simulink model "Controller"  (R2026b)
settings: Solver=VariableStepAuto  StopTime=1200  MaxStep=0.1
values from neighbouring files (symbols this model uses):
  Hoffch = 0.5    [export_ref.m]    (also in init_params.m = 3; testseq.m)
  Honch = 0.5    [export_ref.m]    (also in init_params.m = 3; testseq.m)
  Kich = 6    [init_params.m]
  Kpch = 3000    [init_params.m]
  Ktch = 0.005    [init_params.m]
  Qmax = 24000    [init_params.m]
  Qmin = Qmax/turndown    (= 2400)    [init_params.m]
  Tsch = 0.1    [init_params.m]
undefined symbols (not defined in the file or in its folder): Kbch
libraries: slpidlib x1
settings Model: Creator=Ogun Serif  LastModifiedBy=Ogun Serif
settings DataIOCC: SaveOutput=off  SaveTime=off

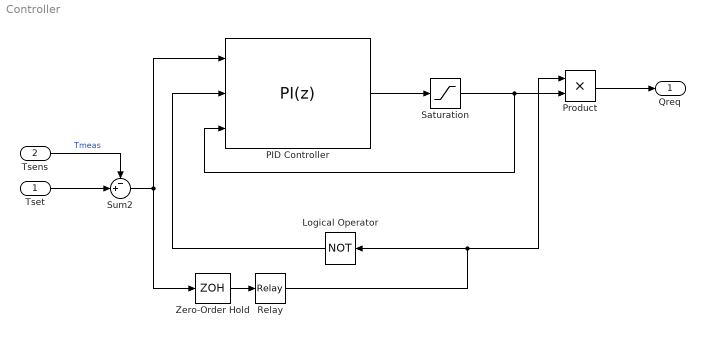
== system Controller ==
  Tset : Inport  OutDataTypeStr=double  PortDimensions=1
  Tsens : Inport  Port=2  OutDataTypeStr=double  PortDimensions=1  SampleTime=0
  Logical Operator : Logic  Operator=NOT  AllPortsSameDT=off  OutDataTypeStr=boolean
  PID Controller : slpidlib/PID Controller  Controller=PI  Form=Parallel  TimeDomain=Discrete-time  UseExternalTs=off  SampleTime=Tsch  IntegratorMethod=Forward Euler  FilterMethod=Forward Euler  ControllerParametersSource=internal  P=Kpch  I=Kich  UseKiTs=off  D=0  UseExternalDerivativeSource=off  N=100  UseFilter=on  TunerSelectOption=Transfer Function Based (PID Tuner App)  InitialConditionSource=internal  InitialConditionForIntegrator=0  InitialConditionForFilter=0  DifferentiatorICPrevScaledInput=0  ExternalReset=level  TrackingMode=on  Kt=Ktch  LimitOutput=off  SatLimitsSource=internal  UpperSaturationLimit=24000  LowerSaturationLimit=Qmin  LinearizeAsGain=on  AntiWindupMode=back-calculation  Kb=Kbch  LimitIntegrator=off  UpperIntegratorSaturationLimit=inf  LowerIntegratorSaturationLimit=-inf  POutMin=[]  POutMax=[]  IOutMin=[]  IOutMax=[]  DOutMin=[]  DOutMax=[]  NOutMin=[]  NOutMax=[]  SumOutMin=[]  SumOutMax=[]  SaturationOutMin=[]  SaturationOutMax=[]  PParamMin=[]  PParamMax=[]  IParamMin=[]  IParamMax=[]  DParamMin=[]  DParamMax=[]  NParamMin=[]  NParamMax=[]  KbParamMin=[]  KbParamMax=[]  KtParamMin=[]  KtParamMax=[]  KbOutMin=[]  KbOutMax=[]  KtOutMin=[]  KtOutMax=[]  IntegratorOutMin=[]  IntegratorOutMax=[]  FilterOutMin=[]  FilterOutMax=[]  SumI1OutMin=[]  SumI1OutMax=[]  SumI2OutMin=[]  SumI2OutMax=[]  SumI3OutMin=[]  SumI3OutMax=[]  SumI4OutMin=[]  SumI4OutMax=[]  SumDOutMin=[]  SumDOutMax=[]  DifferentiatorOutMin=[]  DifferentiatorOutMax=[]  FilterDiffOutCoefMin=[]  FilterDiffOutCoefMax=[]  ReciprocalOutMin=[]  ReciprocalOutMax=[]  SumDenOutMin=[]  SumDenOutMax=[]  SumNumOutMin=[]  SumNumOutMax=[]  DivideOutMin=[]  DivideOutMax=[]  UdiffTsProdOutMin=[]  UdiffTsProdOutMax=[]  NTsProdOutMin=[]  NTsProdOutMax=[]  UintegralTsProdOutMin=[]  UintegralTsProdOutMax=[]  UngainTsProdOutMin=[]  UngainTsProdOutMax=[]  ClampingZeroOutDataTypeStr=Inherit: Inherit via back propagation  ClampingZeroOutMin=[]  ClampingZeroOutMax=[]  FilterDenConstantOutDataTypeStr=Inherit: Inherit via back propagation  FilterDenConstantOutMin=[]  FilterDenConstantOutMax=[]  PCopyOutDataTypeStr=Inherit: Inherit via back propagation  PCopyOutMin=[]  PCopyOutMax=[]  NCopyOutDataTypeStr=Inherit: Inherit via back propagation  NCopyOutMin=[]  NCopyOutMax=[]  IntegratorContinuousStateAttributes=''  IntegratorStateMustResolveToSignalObject=off  IntegratorRTWStateStorageClass=Auto  FilterContinuousStateAttributes=''  FilterStateMustResolveToSignalObject=off  FilterRTWStateStorageClass=Auto  ParallelPVariant=InternalParameters  IdealPVariant=Disabled  IVariant=InternalParameters  DVariant=Disabled  IntegratorVariant=Discrete  SatVariant=Disabled  AWVariant=Passthrough  PCopyVariant=Disabled  TRVariant=Enabled  FdbkBlocksVariant=Forward  IdealPFdbkVariant=Disabled  SatFdbkVariant=Disabled  DerivativeFilterVariant=Disabled  NVariant=Disabled  NCopyVariant=Disabled_SignalSpec  FilterICVariant=Disabled  IntegratorICVariant=InternalICs  ExternalResetVariant=ExternalReset  TRSumVariant=TrackingMode  SumFdbkVariant=Disabled  SumVariant=Sum_PI  TsampFilterVariant=InternalTs  TsampNgainVariant=Passthrough  TsampIntegralVariant=Disabled_SignalSpec  ExternalSaturationOutDataTypeStr=Inherit: Same as second input  DerivativeSourceVariant=Disabled  PreIntVariant=InternalPreInt
  Product : Product
  Relay : Relay  OnSwitchValue=Honch  OffSwitchValue=-Hoffch
  Saturation : Saturate  UpperLimit=Qmax  LowerLimit=Qmin
  Sum2 : Sum  Inputs=-+|
  Zero-Order Hold : ZeroOrderHold  SampleTime=Tsch
  Qreq : Outport  OutDataTypeStr=double  PortDimensions=1  SampleTime=[0.10000000000000001,0]
  wires:
  Sum2/1 -> PID Controller/1, Zero-Order Hold/1
  Tset/1 -> Sum2/2
  PID Controller/1 -> Saturation/1
  Tsens/1 -> Sum2/1  "Tmeas"
  Relay/1 -> Product/1, Logical Operator/1
  Logical Operator/1 -> PID Controller/2
  Saturation/1 -> PID Controller/3, Product/2
  Product/1 -> Qreq/1
  Zero-Order Hold/1 -> Relay/1
